simulink model "EV6_LUT_FourWheel_EV6Battery77p4kWh_PowerCorrected"  (R2024a)
settings: Solver=ode4  StartTime=0  StopTime=60  FixedStep=0.001  RelTol=1e-3
PreLoadFcn:
  | VSS_BICYCLE=Simulink.Variant('Dual=0');
  | VSS_DUAL=Simulink.Variant('Dual=1');
  | Dual=1;
  | load('DriveCycle2.mat')
PostLoadFcn:
  | if any(exist('dsrtsu_mdlpostloadfcn', 'file') ~= 0), dsrtsu_mdlpostloadfcn('Execute', bdroot); end
InitFcn:
  | , if any(exist('rtifpga_mdlclblib', 'file') ~= 0), rtifpga_mdlclblib('Init', bdroot); end,
  | , if any(exist('dsmpb_private', 'file') ~= 0), dsmpb_private('dsmpb_mdlclblib', 'Init', bdroot); end,
  | load('DriveCycle2.mat')
model workspace (MAT data in the model file):
  DiffRatio = 10.65
  EV6_2023_BattBranchCapacity_Ah = 55.5236728838
  EV6_2023_BattEnergy_kWh = 77.4
  EV6_2023_BattNominalVoltage_V = 697
  EV6_2023_BattNumCellsParallel = 2
  EV6_2023_BattNumCellsSeries = 192
  EV6_2023_BattOpenVoltCapBpts = [0 0.1 0.2 0.3 0.4 0.5 0.6 0.7 0.8 0.9 1]
  EV6_2023_BattOpenVoltTbl = [2.96762142548 3.40364281191 3.47417488548 3.54470541822 3.61523441014 3.68576186124 3.75628777151 3.82681214095 3.94527005036 4.07101207308 4.2120755254]
  EV6_2023_BattPackCapacity_Ah = 111.047345768
  EV6_2023_BattResistSocBpts = [0 0.2 0.4 0.6 0.8 1]
  EV6_2023_BattResistTbl = [0.0163620057716 0.0118174152018 0.00807187352333 0.00375663957972 0.00266904525531 0.00103635901355 0.0019014404175 0.0172368903217 0.0121226074867 0.00758541551769 0.00474065349228 0.00337561163613 ... (42 elements, 7x6)]
  EV6_2023_BattResistTempBpts = [243.1 253.1 263.1 273.1 283.1 298.1 313.1]
  EV6_2023_InitialPackOCV_V = 726.471714233
  EV6_2023_InitialSOC = 0.638878863672
  EV6_BattCellCapacity_Ah = 60.3
  EV6_BattInitialSOC = 0.638878863672
  EV6_BattOCV_Cell_V = [2.96762142548 3.40364281191 3.47417488548 3.54470541822 3.61523441014 3.68576186124 3.75628777151 3.82681214095 3.94527005036 4.07101207308 4.2120755254]
  EV6_BattOCV_SOC = [0 0.1 0.2 0.3 0.4 0.5 0.6 0.7 0.8 0.9 1]
  EV6_BattPackCapacity_Ah = 120.6
  EV6_BattParallelCells = 2
  EV6_BattResistanceSOC = [0 0.2 0.4 0.6 0.8 1]
  EV6_BattResistanceTable_Ohm = [0.0163620057716 0.0118174152018 0.00807187352333 0.00375663957972 0.00266904525531 0.00103635901355 0.0019014404175 0.0172368903217 0.0121226074867 0.00758541551769 0.00474065349228 0.00337561163613 ... (42 elements, 7x6)]
  EV6_BattResistanceTemp_K = [243.1 253.1 263.1 273.1 283.1 298.1 313.1]
  EV6_BattSeriesCells = 192
  EV6_FinalDriveRatio = 10.65
  EV6_TargetPackResistance_Ohm = 0.132763804608
  Gas = 0.383333333333
undefined symbols (not defined in the file): accel_bp_mps2, AccelCmd, ActTqLF_Nm_, ActTqLR_Nm_, ActTqRF_Nm_, ActTqRR_Nm_, BattChargeLimitMaxPwr, BattChargeLimitSocBpts, BattChargeLimitTbl, BattDischargeLimitSocBpts, BattDischargeLimitTbl, BattDischargeMaxPwr, BrakeMaxPrs, BrakeMaxTrq, ChassisDistCg2FrontAxle, ChassisDistCg2RearAxle, ChassisVehMass, CltchCmd, CoastDown, DecelCmd, DiscIntNeverNeededParam, EnvGravCnst, EnvPrs, EnvTemp, EV6_RegenTorqueGain, EV6_TractionTorqueGain, front_share_regen_3d, front_share_traction_3d, FuelSpecificGrav, GearCmd, h, InitStates, lgSw, limitedMCT, MCT, MtrEffSpdBpts, MtrEffTbl, MtrEffTrqBpts, MtrPwrMax, MtrTrqMax, out_1, pMCT, RealSimPara, Ref_speed, Ref_time, regen_torque_bp_Nm, speed_bp_kph, SteeringCmd, SupvsryCtrlRegenBrkCutOffTbl, SupvsryCtrlRegenSpdBpts, TestScnrioCycleNum, traction_torque_bp_Nm, US06, VEH
libraries: VSIGenLib x65, simulink x54, etargetslib x38, dsmpblib x24, vehdynlibtire x12, autolibshared x11, vehdynlibsuspension x7, vehdynlibtirecommon x7, autolibpowerinfoutils x6, autolibutils x5, autolibsharedcoupling x4, autolibmappedmotor x4
(part 4 of 19)

== system EV6_LUT_FourWheel_EV6Battery77p4kWh_PowerCorrected/Vehicle Under Test1/Vehicle/Motor_F ==
  SupvsryCtrl : Inport
  MtrSpd : Inport  Port=2
  Bus Creator1 : BusCreator  Inputs=1
  Bus Creator2 : BusCreator  Inputs=4
  Bus Selector1 : BusSelector  OutputSignals=Volt
  Bus Selector2 : BusSelector  OutputSignals=MtrTrqCmd
  Bus Selector3 : BusSelector  OutputSignals=PwrInfo.PwrTrnsfrd.PwrMtr,PwrInfo.PwrTrnsfrd.PwrBus
  Mach-E Motor : autolibmappedmotor/Mapped Motor  port_config=Speed  param_by=Maximum torque and power  w_t=[ 0 375 750 800 ]  T_t=[0.09 0.08 0.07 0]  torque_max=800  power_max=358000  Tc=0.01  param_loss=Tabulated efficiency data  eff=100  w_eff=375  T_eff=0.08  Piron=0  Pbase=0  w_eff_bp=MtrEffSpdBpts.*pi/30  T_eff_bp=MtrEffTrqBpts  Temp_eff_bp=[233.15 293.15 373.15]  losses_table=[1 2;3 4]  losses_table_3d=cat(3,[1.49 1.67 2.21 3.10; 0.42 0.69 1.14 2.03; 0.06 0.24 0.78 1.68; 0.42 0.69 1.14 2.03; 1.49 1.67 2.21 3.10],[1.49 1.67 2.21 3.10; 0.42 0.69 1.14 2.03; 0.06 0.24 0.78 1.68; 0.42 0.69 1.14 2.03; 1.49 1.67 2.21 3.10],[1.49 1.67 2.21 3.10; 0.42 0.69 1.14 2.03; 0.06 0.24 0.78 1.68; 0.42 0.69 1.14 2.03; 1.49 1.67 2.21 3.10])  efficiency_table=MtrEffTbl*0.94  efficiency_table_3d=cat(3,[95 95 95 95; 95 95 95 95; 95 95 95 95; 95 95 95 95; 95 95 95 95],[95 95 95 95; 95 95 95 95; 95 95 95 95; 95 95 95 95; 95 95 95 95],[95 95 95 95; 95 95 95 95; 95 95 95 95; 95 95 95 95; 95 95 95 95])  J=5e-6  b=1e-5  omega_o=0  T_t_extended=[0 0.07 0.08 0.09 0.08 0.07 0]  w_t_extended=[-800 -750 -375 0 375 750 800]  KLossIron=0  KLossCopper=0  x_w_eff_vec=[-1047.1975511966 -942.477796076938 -837.758040957278 -733.038285837618 -628.318530717959 -523.598775598299 -418.879020478639 -314.159265358979 -285.714285713875 -209.43951023932 -104.71975511966 0 104.71975511966 209.43951023932 285.714285713875 314.159265358979 418.879020478639 523.598775598299 628.318530717959 733.038285837618 837.758040957278 942.477796076938 1047.1975511966]  x_T_eff_vec=[-360 -334.285714285714 -308.571428571429 -282.857142857143 -257.142857142857 -231.428571428571 -205.714285714286 -180 -154.285714285714 -128.571428571429 -102.857142857143 -77.1428571428572 -51.4285714285714 -25.7142857142857 0 25.7142857142857 51.4285714285714 77.1428571428572 102.857142857143 128.571428571429 154.285714285714 180 205.714285714286 231.428571428571 257.142857142857 282.857142857143 308.571428571429 334.285714285714 360]  x_tmp_eff_vec=[-0.09 -0.06 -0.03 0 0.03 0.06 0.09]  x_losses_mat=[54250.1517943165 50375.1409518653 46500.1301094142 42625.119266963 38750.1084245118 34875.0975820605 31000.0867396095 27125.0758971582 23250.065054707 19375.054212256 15500.0433698047 12629.4764797412 9803.55154311708 6774.11181875432 0 5412.5153431847 8293.80460547705 10921.9712596802 13550.1379138833 16937.6723923542 20325.2068708249 23712.7413492957 27100.2758277666 30487.8103062373 33875.3447847082 37262.879263179 40650.4137416499 44037.9482201206 47425.4826985915;44696.230836134 41503.6429192672 38311.0550024006 35118.4670855338 31925.8791686671 28733.2912518003 25540.7033349337 22348.115418067 19155.5275012002 15962.9395843336 12770.3516674669 9577.76375060014 6975.01951641212 6096.70063687888 0 4871.26380886623 6097.56206124747 8462.91205003029 11283.8827333737 14104.8534167172 16925.8241000605 19746.794783404 22567.7654667475 25388.7361500908 28209.7068334343 31030.6775167777 33851.6482001212 36672.6188834645 39493.589566808;36137.1105685043 33555.8883850397 30974.6662015752 28393.4440181105 25812.2218346459 23230.9996511813 20649.7774677168 18068.5552842522 15487.3331007875 12906.110917323 10324.8887338584 8513.56777831124 6200.01734792188 5419.28945500345 0 4330.01227454776 5420.05516555331 7522.58848891581 9220.12563933554 11525.1570491694 13830.1884590033 16135.2198688372 18440.2512786711 20745.2826885049 23050.3140983388 25355.3455081727 27660.3769180066 29965.4083278404 32270.4397376744;31619.9717474413 29361.4023369097 27102.8329263783 24844.2635158467 22585.6941053152 20327.1246947836 18068.5552842522 15809.9858737206 13551.4164631891 11292.8470526576 9034.27764212609 7449.37180602233 5425.01517943165 4741.87827312802 0 3788.76074022929 4742.54826985915 6582.26492780134 8067.6099344186 10084.5124180233 12101.4149016279 14118.3173852325 16135.2198688372 18152.1223524418 20169.0248360465 22185.9273196511 24202.8298032558 26219.7322868604 28236.6347704651;27102.8329263782 25166.9162887798 23230.9996511814 21295.0830135829 19359.1663759844 17423.249738386 15487.3331007876 13551.4164631891 11615.4998255906 9679.58318799226 8513.56777831124 6385.17583373343 4650.01301094141 4064.46709125259 0 3247.50920591082 4065.04137416498 5641.94136668686 7522.58848891582 8643.86778687709 10372.6413442524 12101.4149016279 13830.1884590033 15558.9620163787 17287.7355737541 19016.5091311295 20745.282688505 22474.0562458803 24202.8298032558;22585.6941053152 20972.4302406498 19359.1663759845 17745.9025113191 16132.6386466537 14519.3747819883 12906.110917323 11292.8470526576 9679.58318799221 8066.31932332688 7094.63981525937 5320.97986144452 3875.01084245118 3387.05590937716 0 2706.25767159235 3387.53447847082 4701.61780557238 6268.82374076318 7203.22315573091 8643.86778687704 10084.5124180232 11525.1570491694 12965.8016803156 14406.4463114618 15847.0909426079 17287.7355737541 18728.3802049003 20169.0248360465;19864.9914827262 18446.0635196743 17027.1355566225 15608.2075935706 14189.2796305187 12770.3516674668 11351.423704415 9932.4957413631 8513.56777831121 7094.63981525938 5675.71185220749 4256.78388915562 3100.00867396094 2709.64472750173 0 2165.00613727388 2710.02758277665 3761.29424445791 5015.05899261055 6268.82374076319 7522.58848891579 8776.35323706844 10030.1179852211 11283.8827333737 12537.6474815263 13791.412229679 15045.1769778316 16298.9417259842 17552.7064741369;20587.4582405459 19116.9255090783 17646.3927776108 16175.8600461432 12629.4764797412 11366.528831767 10103.581183793 8137.52276914747 6975.01951641211 5812.51626367679 4650.01301094142 3788.84294392236 2525.89529594824 2032.23354562629 0 1623.75460295541 2184.39425193603 3276.59137790406 4065.04137416499 5081.30171770625 6097.56206124746 7113.82240478872 8737.57700774416 9829.77413371214 10921.9712596802 13684.7775990372 14928.8482898587 16172.9189806802 17416.9896715018;18723.4042552922 17386.0182370571 16048.6322188219 14711.2462005868 11485.9634880614 10337.3671392553 9188.77079044916 8040.174441643 6891.57809283685 5742.98174403074 4594.38539522458 ...(+6536 chars)]  x_losses_mat_3d=[37.8947368421052 25.2631578947368 12.6315789473684 0 12 24 36;18.9473684210526 12.6315789473684 6.3157894736842 0 5.99999999999999 12 18;0 0 0 0 0 0 0;18 12 5.99999999999999 0 6.3157894736842 12.6315789473684 18.9473684210526;36 24 12 0 12.6315789473684 25.2631578947368 37.8947368421052]  CalLossMapData={}  CalLossWithTempMapData={}  aMode=aMode  RefBlkName='autolibmappedmotor/Mapped Motor'
  Mapped Motor : autolibmappedmotor/Mapped Motor  port_config=Speed  param_by=Maximum torque and power  w_t=[ 0 375 750 800 ]  T_t=[0.09 0.08 0.07 0]  torque_max=MtrTrqMax  power_max=MtrPwrMax  Tc=MtrTrqTimeCnst  param_loss=Tabulated efficiency data  eff=100  w_eff=375  T_eff=0.08  Piron=0  Pbase=0  w_eff_bp=MtrEffSpdBpts.*pi/30  T_eff_bp=MtrEffTrqBpts  Temp_eff_bp=[233.15 293.15 373.15]  losses_table=[1 2;3 4]  losses_table_3d=cat(3,[1.49 1.67 2.21 3.10; 0.42 0.69 1.14 2.03; 0.06 0.24 0.78 1.68; 0.42 0.69 1.14 2.03; 1.49 1.67 2.21 3.10],[1.49 1.67 2.21 3.10; 0.42 0.69 1.14 2.03; 0.06 0.24 0.78 1.68; 0.42 0.69 1.14 2.03; 1.49 1.67 2.21 3.10],[1.49 1.67 2.21 3.10; 0.42 0.69 1.14 2.03; 0.06 0.24 0.78 1.68; 0.42 0.69 1.14 2.03; 1.49 1.67 2.21 3.10])  efficiency_table=MtrEffTbl*0.94  efficiency_table_3d=cat(3,[95 95 95 95; 95 95 95 95; 95 95 95 95; 95 95 95 95; 95 95 95 95],[95 95 95 95; 95 95 95 95; 95 95 95 95; 95 95 95 95; 95 95 95 95],[95 95 95 95; 95 95 95 95; 95 95 95 95; 95 95 95 95; 95 95 95 95])  J=5e-6  b=1e-5  omega_o=0  T_t_extended=[0 0.07 0.08 0.09 0.08 0.07 0]  w_t_extended=[-800 -750 -375 0 375 750 800]  KLossIron=0  KLossCopper=0  x_w_eff_vec=[-1047.1975511966 -942.477796076938 -837.758040957278 -733.038285837618 -628.318530717959 -523.598775598299 -418.879020478639 -314.159265358979 -285.714285713875 -209.43951023932 -104.71975511966 0 104.71975511966 209.43951023932 285.714285713875 314.159265358979 418.879020478639 523.598775598299 628.318530717959 733.038285837618 837.758040957278 942.477796076938 1047.1975511966]  x_T_eff_vec=[-360 -334.285714285714 -308.571428571429 -282.857142857143 -257.142857142857 -231.428571428571 -205.714285714286 -180 -154.285714285714 -128.571428571429 -102.857142857143 -77.1428571428572 -51.4285714285714 -25.7142857142857 0 25.7142857142857 51.4285714285714 77.1428571428572 102.857142857143 128.571428571429 154.285714285714 180 205.714285714286 231.428571428571 257.142857142857 282.857142857143 308.571428571429 334.285714285714 360]  x_tmp_eff_vec=[-0.09 -0.06 -0.03 0 0.03 0.06 0.09]  x_losses_mat=[54250.1517943165 50375.1409518653 46500.1301094142 42625.119266963 38750.1084245118 34875.0975820605 31000.0867396095 27125.0758971582 23250.065054707 19375.054212256 15500.0433698047 12629.4764797412 9803.55154311708 6774.11181875432 0 5412.5153431847 8293.80460547705 10921.9712596802 13550.1379138833 16937.6723923542 20325.2068708249 23712.7413492957 27100.2758277666 30487.8103062373 33875.3447847082 37262.879263179 40650.4137416499 44037.9482201206 47425.4826985915;44696.230836134 41503.6429192672 38311.0550024006 35118.4670855338 31925.8791686671 28733.2912518003 25540.7033349337 22348.115418067 19155.5275012002 15962.9395843336 12770.3516674669 9577.76375060014 6975.01951641212 6096.70063687888 0 4871.26380886623 6097.56206124747 8462.91205003029 11283.8827333737 14104.8534167172 16925.8241000605 19746.794783404 22567.7654667475 25388.7361500908 28209.7068334343 31030.6775167777 33851.6482001212 36672.6188834645 39493.589566808;36137.1105685043 33555.8883850397 30974.6662015752 28393.4440181105 25812.2218346459 23230.9996511813 20649.7774677168 18068.5552842522 15487.3331007875 12906.110917323 10324.8887338584 8513.56777831124 6200.01734792188 5419.28945500345 0 4330.01227454776 5420.05516555331 7522.58848891581 9220.12563933554 11525.1570491694 13830.1884590033 16135.2198688372 18440.2512786711 20745.2826885049 23050.3140983388 25355.3455081727 27660.3769180066 29965.4083278404 32270.4397376744;31619.9717474413 29361.4023369097 27102.8329263783 24844.2635158467 22585.6941053152 20327.1246947836 18068.5552842522 15809.9858737206 13551.4164631891 11292.8470526576 9034.27764212609 7449.37180602233 5425.01517943165 4741.87827312802 0 3788.76074022929 4742.54826985915 6582.26492780134 8067.6099344186 10084.5124180233 12101.4149016279 14118.3173852325 16135.2198688372 18152.1223524418 20169.0248360465 22185.9273196511 24202.8298032558 26219.7322868604 28236.6347704651;27102.8329263782 25166.9162887798 23230.9996511814 21295.0830135829 19359.1663759844 17423.249738386 15487.3331007876 13551.4164631891 11615.4998255906 9679.58318799226 8513.56777831124 6385.17583373343 4650.01301094141 4064.46709125259 0 3247.50920591082 4065.04137416498 5641.94136668686 7522.58848891582 8643.86778687709 10372.6413442524 12101.4149016279 13830.1884590033 15558.9620163787 17287.7355737541 19016.5091311295 20745.282688505 22474.0562458803 24202.8298032558;22585.6941053152 20972.4302406498 19359.1663759845 17745.9025113191 16132.6386466537 14519.3747819883 12906.110917323 11292.8470526576 9679.58318799221 8066.31932332688 7094.63981525937 5320.97986144452 3875.01084245118 3387.05590937716 0 2706.25767159235 3387.53447847082 4701.61780557238 6268.82374076318 7203.22315573091 8643.86778687704 10084.5124180232 11525.1570491694 12965.8016803156 14406.4463114618 15847.0909426079 17287.7355737541 18728.3802049003 20169.0248360465;19864.9914827262 18446.0635196743 17027.1355566225 15608.2075935706 14189.2796305187 12770.3516674668 11351.423704415 9932.4957413631 8513.56777831121 7094.63981525938 5675.71185220749 4256.78388915562 3100.00867396094 2709.64472750173 0 2165.00613727388 2710.02758277665 3761.29424445791 5015.05899261055 6268.82374076319 7522.58848891579 8776.35323706844 10030.1179852211 11283.8827333737 12537.6474815263 13791.412229679 15045.1769778316 16298.9417259842 17552.7064741369;20587.4582405459 19116.9255090783 17646.3927776108 16175.8600461432 12629.4764797412 11366.528831767 10103.581183793 8137.52276914747 6975.01951641211 5812.51626367679 4650.01301094142 3788.84294392236 2525.89529594824 2032.23354562629 0 1623.75460295541 2184.39425193603 3276.59137790406 4065.04137416499 5081.30171770625 6097.56206124746 7113.82240478872 8737.57700774416 9829.77413371214 10921.9712596802 13684.7775990372 14928.8482898587 16172.9189806802 17416.9896715018;18723.4042552922 17386.0182370571 16048.6322188219 14711.2462005868 11485.9634880614 10337.3671392553 9188.77079044916 8040.174441643 6891.57809283685 5742.98174403074 4594.38539522458 ...(+6536 chars)]  x_losses_mat_3d=[37.8947368421052 25.2631578947368 12.6315789473684 0 12 24 36;18.9473684210526 12.6315789473684 6.3157894736842 0 5.99999999999999 12 18;0 0 0 0 0 0 0;18 12 5.99999999999999 0 6.3157894736842 12.6315789473684 18.9473684210526;36 24 12 0 12.6315789473684 25.2631578947368 37.8947368421052]  CalLossMapData={}  CalLossWithTempMapData={}  aMode=aMode  RefBlkName='autolibmappedmotor/Mapped Motor'
  Memory : Memory
  Mux{,1..3} (4 alike) : Mux  Inputs=1
  Scope : Scope
  To Workspace : ToWorkspace  VariableName=MtrTrq_F_Mache  SaveFormat=Structure With Time  SampleTime=-1
  Two-Way Connection1 : TwoWayConnection
  Batt : PMIOPort  Side=Left
  Mtr : Outport
  MtrTrq : Outport  Port=2
  wires:
  Mach-E Motor/3 -> Mux/1, MtrTrq/1, To Workspace/1  "Trq"
  Mach-E Motor/2 -> Memory/1  "Curr"
  Bus Creator1/1 -> Two-Way Connection1/1
  Mach-E Motor/1 -> Bus Selector3/1
  SupvsryCtrl/1 -> Bus Selector2/1
  Two-Way Connection1/1 -> Bus Selector1/1
  Bus Selector1/1 -> Mach-E Motor/1  "<Volt>"
  Bus Selector2/1 -> Scope/1, Mach-E Motor/3  "<MtrTrqCmd>"
  Mux/1 -> Bus Creator2/2  "MtrTrq"
  Bus Creator2/1 -> Mtr/1
  Mux2/1 -> Bus Creator2/3  "MtrMechPwr"
  Bus Selector3/1 -> Mux2/1  "<PwrMtr>"
  Mux1/1 -> Bus Creator2/1  "MtrSpd"
  Bus Selector3/2 -> Mux3/1  "<PwrBus>"
  Mux3/1 -> Bus Creator2/4  "MtrElecPwr"
  Memory/1 -> Bus Creator1/1  "Curr"
  MtrSpd/1 -> Mach-E Motor/2, Mux1/1
  connections:
  Batt/RConn1 -- Two-Way Connection1/RConn1
